simulink model "BESS_ctrl"  (R2026a)
settings: Solver=FixedStepDiscrete  StopTime=inf  FixedStep=Ts
model workspace (MATLAB code in the model file):
  | % Defaults for standalone use and code generation, from HPP_parameters.
  | % In HPP.slx the Model block passes p.ctrl.bess.par as the argument "par".
  | pDefault = HPP_parameters();
  | Ts  = pDefault.ctrl.bess.Ts;    % [s] fixed sample time
  | par = pDefault.ctrl.bess.par;   % tunable parameters (model argument)
  | clear pDefault
libraries: simulink x3, slpidlib x1, sl_discontinuities x1
Description:
  | BESS asset controller: WECC REEC_C electrical control (voltage filter and dip detection, P path with ramp and Tpord lag, Q path with Qflag (closed-loop Q PI) and dip current injection Kqv, current limit logic with PQflag, state-of-charge limits). Per unit on the asset rating. Parameters: model argument par (= p.ctrl.bess.par, from p.bess.wecc.ctrl). Simplified; details and values to be checked against the WECC specification.
settings Model: ParameterArgumentNames=par  Creator=kjaer  LastModifiedBy=kjaer

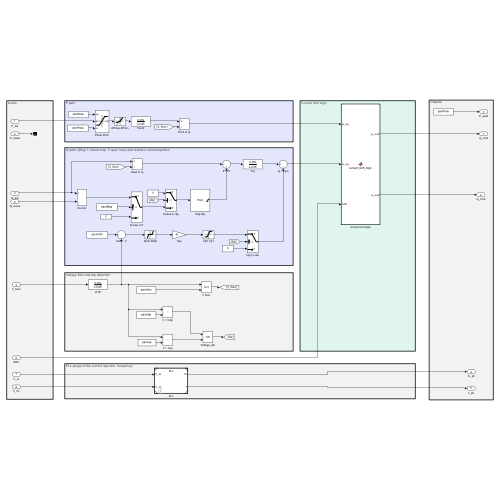
[thumbnail: Simulink's stored preview of the top-level diagram]
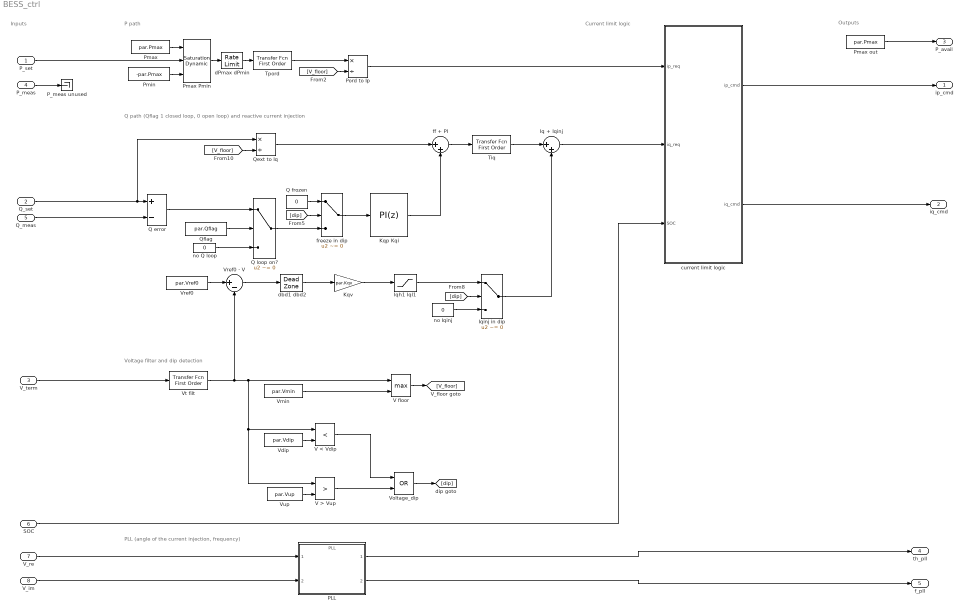
== system BESS_ctrl ==
  note: Voltage filter and dip detection
  note: Outputs
  note: PLL (angle of the current injection, frequency)
  note: Current limit logic
  note: Q path (Qflag 1 closed loop, 0 open loop) and reactive current injection
  note: P path
  note: Inputs
  P_set : Inport  OutDataTypeStr=double  PortDimensions=1  SampleTime=Ts
  Q_set : Inport  Port=2  OutDataTypeStr=double  PortDimensions=1  SampleTime=Ts
  V_term : Inport  Port=3  OutDataTypeStr=double  PortDimensions=1  SampleTime=Ts
  P_meas : Inport  Port=4  OutDataTypeStr=double  PortDimensions=1  SampleTime=Ts
  Q_meas : Inport  Port=5  OutDataTypeStr=double  PortDimensions=1  SampleTime=Ts
  SOC : Inport  Port=6  OutDataTypeStr=double  PortDimensions=1  SampleTime=Ts
  V_re : Inport  Port=7  OutDataTypeStr=double  PortDimensions=1  SampleTime=Ts
  V_im : Inport  Port=8  OutDataTypeStr=double  PortDimensions=1  SampleTime=Ts
  Iq + Iqinj : Sum  Inputs=|++
  Iqh1 Iql1 : Saturate  UpperLimit=par.Iqh1  LowerLimit=par.Iql1
  Iqinj in dip : Switch  Criteria=u2 ~= 0  SaturateOnIntegerOverflow=off  InputSameDT=off
  Kqp Kqi : slpidlib/PID Controller  Controller=PI  Form=Parallel  TimeDomain=Discrete-time  UseExternalTs=off  SampleTime=-1  IntegratorMethod=Forward Euler  FilterMethod=Forward Euler  ControllerParametersSource=internal  P=par.Kqp  I=par.Kqi  UseKiTs=off  D=0  UseExternalDerivativeSource=off  N=100  UseFilter=on  TunerSelectOption=Transfer Function Based (PID Tuner App)  InitialConditionSource=internal  InitialConditionForIntegrator=0  InitialConditionForFilter=0  DifferentiatorICPrevScaledInput=0  ExternalReset=none  TrackingMode=off  Kt=1  LimitOutput=on  SatLimitsSource=internal  UpperSaturationLimit=par.Imax  LowerSaturationLimit=-par.Imax  LinearizeAsGain=off  AntiWindupMode=clamping  Kb=1  LimitIntegrator=off  UpperIntegratorSaturationLimit=inf  LowerIntegratorSaturationLimit=-inf  POutMin=[]  POutMax=[]  IOutMin=[]  IOutMax=[]  DOutMin=[]  DOutMax=[]  NOutMin=[]  NOutMax=[]  SumOutMin=[]  SumOutMax=[]  SaturationOutMin=[]  SaturationOutMax=[]  PParamMin=[]  PParamMax=[]  IParamMin=[]  IParamMax=[]  DParamMin=[]  DParamMax=[]  NParamMin=[]  NParamMax=[]  KbParamMin=[]  KbParamMax=[]  KtParamMin=[]  KtParamMax=[]  KbOutMin=[]  KbOutMax=[]  KtOutMin=[]  KtOutMax=[]  IntegratorOutMin=[]  IntegratorOutMax=[]  FilterOutMin=[]  FilterOutMax=[]  SumI1OutMin=[]  SumI1OutMax=[]  SumI2OutMin=[]  SumI2OutMax=[]  SumI3OutMin=[]  SumI3OutMax=[]  SumI4OutMin=[]  SumI4OutMax=[]  SumDOutMin=[]  SumDOutMax=[]  DifferentiatorOutMin=[]  DifferentiatorOutMax=[]  FilterDiffOutCoefMin=[]  FilterDiffOutCoefMax=[]  ReciprocalOutMin=[]  ReciprocalOutMax=[]  SumDenOutMin=[]  SumDenOutMax=[]  SumNumOutMin=[]  SumNumOutMax=[]  DivideOutMin=[]  DivideOutMax=[]  UdiffTsProdOutMin=[]  UdiffTsProdOutMax=[]  NTsProdOutMin=[]  NTsProdOutMax=[]  UintegralTsProdOutMin=[]  UintegralTsProdOutMax=[]  UngainTsProdOutMin=[]  UngainTsProdOutMax=[]  ClampingZeroOutDataTypeStr=Inherit: Inherit via back propagation  ClampingZeroOutMin=[]  ClampingZeroOutMax=[]  FilterDenConstantOutDataTypeStr=Inherit: Inherit via back propagation  FilterDenConstantOutMin=[]  FilterDenConstantOutMax=[]  PCopyOutDataTypeStr=Inherit: Inherit via back propagation  PCopyOutMin=[]  PCopyOutMax=[]  NCopyOutDataTypeStr=Inherit: Inherit via back propagation  NCopyOutMin=[]  NCopyOutMax=[]  IntegratorContinuousStateAttributes=''  IntegratorStateMustResolveToSignalObject=off  IntegratorRTWStateStorageClass=Auto  FilterContinuousStateAttributes=''  FilterStateMustResolveToSignalObject=off  FilterRTWStateStorageClass=Auto  ParallelPVariant=InternalParameters  IdealPVariant=Disabled  IVariant=InternalParameters  DVariant=Disabled  IntegratorVariant=Discrete  SatVariant=Enabled  AWVariant=DiscClampingParallel  PCopyVariant=Disabled  TRVariant=Disabled  FdbkBlocksVariant=Forward  IdealPFdbkVariant=Disabled  SatFdbkVariant=Disabled  DerivativeFilterVariant=Disabled  NVariant=Disabled  NCopyVariant=Disabled_SignalSpec  FilterICVariant=Disabled  IntegratorICVariant=InternalICs  ExternalResetVariant=Disabled  TRSumVariant=Passthrough  SumFdbkVariant=Disabled  SumVariant=Sum_PI  TsampFilterVariant=InternalTs  TsampNgainVariant=Passthrough  TsampIntegralVariant=Disabled_SignalSpec  ExternalSaturationOutDataTypeStr=Inherit: Same as second input  DerivativeSourceVariant=Disabled  PreIntVariant=InternalPreInt
      settings: LibrarySourceBlock=simulink/Discrete/Discrete PID Controller
  Kqv : Gain  Gain=par.Kqv
  PLL : ModelReference  ModelNameDialog=PLL  ParameterArgumentNames=pll  ParameterArgumentValues=par.pll  UsingDefaultArgumentValue=0  SimulationMode=Normal  ModelReferenceVersion=1.1
  P_meas unused : Terminator
  Pmax : Constant  Value=par.Pmax
  Pmax Pmin : sl_discontinuities/Saturation Dynamic  OutMin=[]  OutMax=[]  OutDataTypeStr=Inherit: Same as second input  OutDataType=fixdt(1, 16)  OutScaling=2^-10  DoSatur=off
      settings: LibrarySourceBlock=|
      | simulink/Discontinuities/Saturation
      | Dynamic
  Pmax out : Constant  Value=par.Pmax
  Pmin : Constant  Value=-par.Pmax
  Pord to Ip : Product  Inputs=*/
  Q error : Sum  Inputs=+-
  Q frozen : Constant  Value=0
  Q loop on? : Switch  Criteria=u2 ~= 0  SaturateOnIntegerOverflow=off  InputSameDT=off
  Qext to Iq : Product  Inputs=*/
  Qflag : Constant  Value=par.Qflag
  Tiq : simulink/Discrete/Transfer Fcn First Order  PoleZ=1 - Ts/par.Tiq  ICPrevOutput=0  DoSatur=off
  Tpord : simulink/Discrete/Transfer Fcn First Order  PoleZ=1 - Ts/par.Tpord  ICPrevOutput=0  DoSatur=off
  V < Vdip : RelationalOperator  Operator=<  OutDataTypeStr=boolean  RndMeth=Simplest  InputSameDT=off
  V > Vup : RelationalOperator  Operator=>  OutDataTypeStr=boolean  RndMeth=Simplest  InputSameDT=off
  V floor : MinMax  Function=max  Inputs=2
  Vdip : Constant  Value=par.Vdip
  Vmin : Constant  Value=par.Vmin
  Voltage_dip : Logic  Operator=OR  AllPortsSameDT=off  OutDataTypeStr=boolean
  Vref0 : Constant  Value=par.Vref0
  Vref0 - V : Sum  Inputs=|+-
  Vt filt : simulink/Discrete/Transfer Fcn First Order  PoleZ=1 - Ts/par.Trv  ICPrevOutput=1  DoSatur=off
  Vup : Constant  Value=par.Vup
  current limit logic : MATLAB Function  TreatAsAtomicUnit=on
  dPmax dPmin : RateLimiter  RisingSlewLimit=par.dPmax  FallingSlewLimit=par.dPmin  SampleTimeMode=inherited
  dbd1 dbd2 : DeadZone  LowerValue=par.dbd1  UpperValue=par.dbd2
  ff + PI : Sum  Inputs=|++
  freeze in dip : Switch  Criteria=u2 ~= 0  SaturateOnIntegerOverflow=off  InputSameDT=off
  no Iqinj : Constant  Value=0
  no Q loop : Constant  Value=0
  ip_cmd : Outport  OutDataTypeStr=double
  iq_cmd : Outport  Port=2  OutDataTypeStr=double
  P_avail : Outport  Port=3  OutDataTypeStr=double
  th_pll : Outport  Port=4  OutDataTypeStr=double
  f_pll : Outport  Port=5  OutDataTypeStr=double
  wires:
  Tiq/1 -> Iq + Iqinj/1
  Iqh1 Iql1/1 -> Iqinj in dip/1
  Tpord/1 -> Pord to Ip/1
  Qext to Iq/1 -> ff + PI/1
  V > Vup/1 -> Voltage_dip/2
  Vt filt/1 -> Vref0 - V/2, V floor/1, V < Vdip/1, V > Vup/1
  Vmin/1 -> V floor/2
  Q error/1 -> Q loop on?/1
  Vref0/1 -> Vref0 - V/1
  Pord to Ip/1 -> current limit logic/1(ip_req)
  Iqinj in dip/1 -> Iq + Iqinj/2
  Q_meas/1 -> Q error/2
  V_re/1 -> PLL/1
  [V_floor] -> Qext to Iq/2
  [dip] -> Iqinj in dip/2
  SOC/1 -> current limit logic/3(SOC)
  V_term/1 -> Vt filt/1
  [dip] -> freeze in dip/2
  Q_set/1 -> Q error/1, Qext to Iq/1
  [V_floor] -> Pord to Ip/2
  PLL/1 -> th_pll/1
  P_set/1 -> Pmax Pmin/2
  no Q loop/1 -> Q loop on?/3
  no Iqinj/1 -> Iqinj in dip/3
  Iq + Iqinj/1 -> current limit logic/2(iq_req)
  current limit logic/2(iq_cmd) -> iq_cmd/1
  Kqp Kqi/1 -> ff + PI/2
  current limit logic/1(ip_cmd) -> ip_cmd/1
  freeze in dip/1 -> Kqp Kqi/1
  ff + PI/1 -> Tiq/1
  Voltage_dip/1 -> [dip]
  dbd1 dbd2/1 -> Kqv/1
  dPmax dPmin/1 -> Tpord/1
  Vup/1 -> V > Vup/2
  Vref0 - V/1 -> dbd1 dbd2/1
  Vdip/1 -> V < Vdip/2
  V_im/1 -> PLL/2
  V floor/1 -> [V_floor]
  V < Vdip/1 -> Voltage_dip/1
  Qflag/1 -> Q loop on?/2
  Q loop on?/1 -> freeze in dip/3
  Q frozen/1 -> freeze in dip/1
  Pmin/1 -> Pmax Pmin/3
  Pmax out/1 -> P_avail/1
  Pmax Pmin/1 -> dPmax dPmin/1
  Pmax/1 -> Pmax Pmin/1
  P_meas/1 -> P_meas unused/1
  Kqv/1 -> Iqh1 Iql1/1
  PLL/2 -> f_pll/1

== matlab function BESS_ctrl/current limit logic ==
  data: ip_req input; ip_cmd output; iq_req input; SOC input; iq_cmd output; par parameter
function [ip_cmd, iq_cmd] = current_limit_logic(ip_req, iq_req, SOC, par)
%#codegen
% WECC current limit logic (without VDL tables): |I| <= Imax;
% PQflag = 0: Q priority, PQflag = 1: P priority.
% REEC_C: no discharge at SOC <= SOCmin, no charge at SOC >= SOCmax.
ipmin_soc = -par.Imax;  ipmax_soc = par.Imax;
if SOC <= par.SOCmin, ipmax_soc = 0; end
if SOC >= par.SOCmax, ipmin_soc = 0; end
Imax = par.Imax;
if par.PQflag == 0   % Q priority
    iq_cmd = min(max(iq_req, -Imax), Imax);
    ipmax  = sqrt(max(Imax^2 - iq_cmd^2, 0));
    ip_cmd = min(max(ip_req, max(-ipmax, ipmin_soc)), min(ipmax, ipmax_soc));
else                 % P priority
    ip_cmd = min(max(ip_req, max(-Imax, ipmin_soc)), min(Imax, ipmax_soc));
    iqmax  = sqrt(max(Imax^2 - ip_cmd^2, 0));
    iq_cmd = min(max(iq_req, -iqmax), iqmax);
end
end
